simulink library "xps_library"  (Simulink 8.0)
settings: Solver=ode45  SolverMode=SingleTasking  StartTime=0.0  StopTime=10.0  RelTol=1e-3
undefined symbols (not defined in the file): sys_clk, xps_library_software_register_user_data_in
libraries: xbsIndex_r4 x867, simulink x109, dspsigops x81, casper_library_flow_control x68, xps_library x18, casper_library_misc x11
(part 3 of 10)

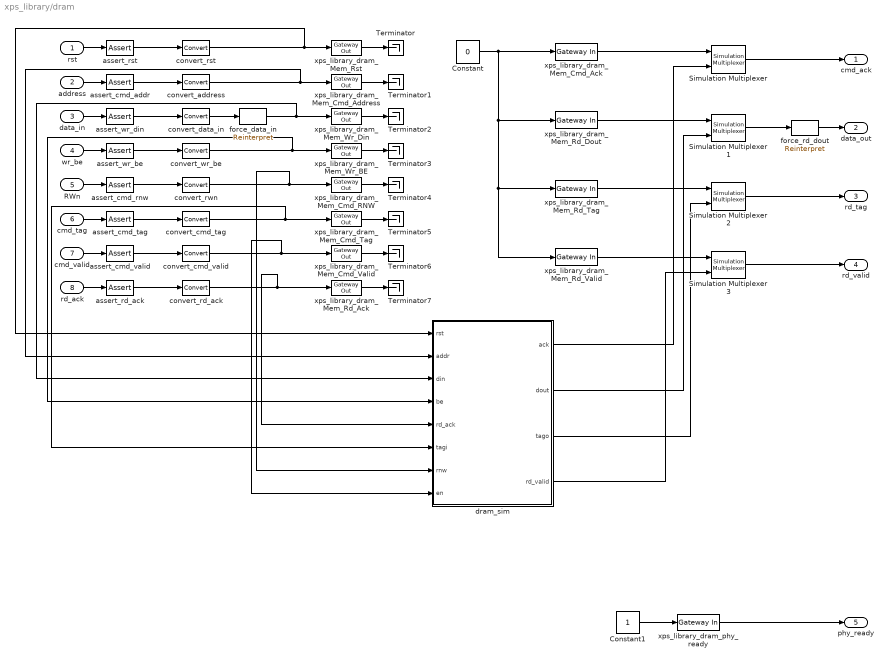
== system xps_library/dram ==
  rst : Inport
  address : Inport  Port=2
  data_in : Inport  Port=3
  wr_be : Inport  Port=4
  RWn : Inport  Port=5
  cmd_tag : Inport  Port=6
  cmd_valid : Inport  Port=7
  rd_ack : Inport  Port=8
  Constant : Constant  Value=0
  Constant1 : Constant
  Simulation Multiplexer{,1..3} (4 alike) : xbsIndex_r4/Simulation Multiplexer  sim_sel=2  hw_sel=1  block_type=simmux
      settings: infoedit="Distinguish input subsystems as \"simulation only\" and \"generation only\".  The input specified For Simulation will be used during Simulink simulation.  The input specified For Generation will be used during code generation.  This block will typically be used on the output of a HW Co-Simulation, Black Box, or ModelSim subsystem.<P><P>Hardware Notes: This block costs nothing."  block_version=9.1.01
  Terminator{,1..7} (8 alike) : Terminator
  assert_cmd_addr : xbsIndex_r4/Assert  assert_type=off  type_source=Explicitly  gui_display_data_type=Fixed-point  arith_type="Signed  (2's comp)"  n_bits=16  bin_pt=14  preci_type=Single  exp_width=8  frac_width=24  assert_rate=on  rate_source=Explicitly  period=sample_period  output_port=on  block_type=assert
      settings: infoedit=Asserts a user-defined sample rate and/or type on a signal.<P><P>Hardware notes: In hardware this block costs nothing.  block_version=9.1.01
  assert_cmd_rnw : xbsIndex_r4/Assert  assert_type=off  type_source=Explicitly  gui_display_data_type=Fixed-point  arith_type="Signed  (2's comp)"  n_bits=16  bin_pt=14  preci_type=Single  exp_width=8  frac_width=24  assert_rate=on  rate_source=Explicitly  period=sample_period  output_port=on  block_type=assert
      settings: infoedit=Asserts a user-defined sample rate and/or type on a signal.<P><P>Hardware notes: In hardware this block costs nothing.  block_version=9.1.01
  assert_cmd_tag : xbsIndex_r4/Assert  assert_type=off  type_source=Explicitly  gui_display_data_type=Fixed-point  arith_type="Signed  (2's comp)"  n_bits=16  bin_pt=14  preci_type=Single  exp_width=8  frac_width=24  assert_rate=on  rate_source=Explicitly  period=sample_period  output_port=on  block_type=assert
      settings: infoedit=Asserts a user-defined sample rate and/or type on a signal.<P><P>Hardware notes: In hardware this block costs nothing.  block_version=9.1.01
  assert_cmd_valid : xbsIndex_r4/Assert  assert_type=off  type_source=Explicitly  gui_display_data_type=Fixed-point  arith_type="Signed  (2's comp)"  n_bits=16  bin_pt=14  preci_type=Single  exp_width=8  frac_width=24  assert_rate=on  rate_source=Explicitly  period=sample_period  output_port=on  block_type=assert
      settings: infoedit=Asserts a user-defined sample rate and/or type on a signal.<P><P>Hardware notes: In hardware this block costs nothing.  block_version=9.1.01
  assert_rd_ack : xbsIndex_r4/Assert  assert_type=off  type_source=Explicitly  gui_display_data_type=Fixed-point  arith_type="Signed  (2's comp)"  n_bits=16  bin_pt=14  preci_type=Single  exp_width=8  frac_width=24  assert_rate=on  rate_source=Explicitly  period=sample_period  output_port=on  block_type=assert
      settings: infoedit=Asserts a user-defined sample rate and/or type on a signal.<P><P>Hardware notes: In hardware this block costs nothing.  block_version=9.1.01
  assert_rst : xbsIndex_r4/Assert  assert_type=off  type_source=Explicitly  gui_display_data_type=Fixed-point  arith_type="Signed  (2's comp)"  n_bits=16  bin_pt=14  preci_type=Single  exp_width=8  frac_width=24  assert_rate=on  rate_source=Explicitly  period=sample_period  output_port=on  block_type=assert
      settings: infoedit=Asserts a user-defined sample rate and/or type on a signal.<P><P>Hardware notes: In hardware this block costs nothing.  block_version=9.1.01
  assert_wr_be : xbsIndex_r4/Assert  assert_type=off  type_source=Explicitly  gui_display_data_type=Fixed-point  arith_type="Signed  (2's comp)"  n_bits=16  bin_pt=14  preci_type=Single  exp_width=8  frac_width=24  assert_rate=on  rate_source=Explicitly  period=sample_period  output_port=on  block_type=assert
      settings: infoedit=Asserts a user-defined sample rate and/or type on a signal.<P><P>Hardware notes: In hardware this block costs nothing.  block_version=9.1.01
  assert_wr_din : xbsIndex_r4/Assert  assert_type=off  type_source=Explicitly  gui_display_data_type=Fixed-point  arith_type="Signed  (2's comp)"  n_bits=16  bin_pt=14  preci_type=Single  exp_width=8  frac_width=24  assert_rate=on  rate_source=Explicitly  period=sample_period  output_port=on  block_type=assert
      settings: infoedit=Asserts a user-defined sample rate and/or type on a signal.<P><P>Hardware notes: In hardware this block costs nothing.  block_version=9.1.01
  convert_address : xbsIndex_r4/Convert  gui_display_data_type=Fixed-point  arith_type=Unsigned  n_bits=32  bin_pt=0  float_type=Single  exp_bits=8  fraction_bits=24  quantization=Truncate  overflow=Wrap  en=off  latency=0  dbl_ovrd=off  pipeline=off  block_type=convert
      settings: xl_area=[0, 0, 0, 0, 0, 0, 0]
  convert_cmd_tag : xbsIndex_r4/Convert  gui_display_data_type=Fixed-point  arith_type=Unsigned  n_bits=32  bin_pt=0  float_type=Single  exp_bits=8  fraction_bits=24  quantization=Truncate  overflow=Wrap  en=off  latency=0  dbl_ovrd=off  pipeline=off  block_type=convert
      settings: xl_area=[0, 0, 0, 0, 0, 0, 0]
  convert_cmd_valid : xbsIndex_r4/Convert  gui_display_data_type=Fixed-point  arith_type=Unsigned  n_bits=1  bin_pt=0  float_type=Single  exp_bits=8  fraction_bits=24  quantization=Truncate  overflow=Wrap  en=off  latency=0  dbl_ovrd=off  pipeline=off  block_type=convert
      settings: xl_area=[0, 0, 0, 0, 0, 0, 0]
  convert_data_in : xbsIndex_r4/Convert  gui_display_data_type=Fixed-point  arith_type=Unsigned  n_bits=144  bin_pt=0  float_type=Single  exp_bits=8  fraction_bits=24  quantization=Truncate  overflow=Wrap  en=off  latency=0  dbl_ovrd=off  pipeline=off  block_type=convert
      settings: xl_area=[0, 0, 0, 0, 0, 0, 0]
  convert_rd_ack : xbsIndex_r4/Convert  gui_display_data_type=Fixed-point  arith_type=Unsigned  n_bits=1  bin_pt=0  float_type=Single  exp_bits=8  fraction_bits=24  quantization=Truncate  overflow=Wrap  en=off  latency=0  dbl_ovrd=off  pipeline=off  block_type=convert
      settings: xl_area=[0, 0, 0, 0, 0, 0, 0]
  convert_rst : xbsIndex_r4/Convert  gui_display_data_type=Fixed-point  arith_type=Unsigned  n_bits=1  bin_pt=0  float_type=Single  exp_bits=8  fraction_bits=24  quantization=Truncate  overflow=Wrap  en=off  latency=0  dbl_ovrd=off  pipeline=off  block_type=convert
      settings: xl_area=[0, 0, 0, 0, 0, 0, 0]
  convert_rwn : xbsIndex_r4/Convert  gui_display_data_type=Fixed-point  arith_type=Unsigned  n_bits=1  bin_pt=0  float_type=Single  exp_bits=8  fraction_bits=24  quantization=Truncate  overflow=Wrap  en=off  latency=0  dbl_ovrd=off  pipeline=off  block_type=convert
      settings: xl_area=[0, 0, 0, 0, 0, 0, 0]
  convert_wr_be : xbsIndex_r4/Convert  gui_display_data_type=Fixed-point  arith_type=Unsigned  n_bits=18  bin_pt=0  float_type=Single  exp_bits=8  fraction_bits=24  quantization=Truncate  overflow=Wrap  en=off  latency=0  dbl_ovrd=off  pipeline=off  block_type=convert
      settings: xl_area=[0, 0, 0, 0, 0, 0, 0]
  dram_sim : Subsystem
  force_data_in : xbsIndex_r4/Reinterpret  force_arith_type=on  arith_type=Unsigned  force_bin_pt=on  bin_pt=0  block_type=reinterpret
      settings: infoedit="Changes signal type without altering the binary representation.   You can changed the signal between signed and unsigned, and relocate the binary point.<P><P>Hardware notes: In hardware this block costs nothing.<P><P>Example:  Suppose the input is 6 bits wide, signed, with 2 fractional bits, and the output is forced to unsigned with 0 fractional bits.  Then an input of -2.0 (1110.00 in binary 2's complement) becomes an output of 56 (111000 in binary)."  block_version=9.1.01
  force_rd_dout : xbsIndex_r4/Reinterpret  force_arith_type=on  arith_type=Unsigned  force_bin_pt=on  bin_pt=0  block_type=reinterpret
      settings: infoedit="Changes signal type without altering the binary representation.   You can changed the signal between signed and unsigned, and relocate the binary point.<P><P>Hardware notes: In hardware this block costs nothing.<P><P>Example:  Suppose the input is 6 bits wide, signed, with 2 fractional bits, and the output is forced to unsigned with 0 fractional bits.  Then an input of -2.0 (1110.00 in binary 2's complement) becomes an output of 56 (111000 in binary)."  block_version=9.1.01
  xps_library_dram_Mem_Cmd_Ack : xbsIndex_r4/Gateway In  gui_display_data_type=Fixed-point  arith_type=Boolean  n_bits=1  bin_pt=0  preci_type=Single  exp_width=8  frac_width=24  quantization=Truncate  overflow=Wrap  period=sample_period  dbl_ovrd=off  timing_constraint=None  locs_specified=off  LOCs={}  hdl_port=on  block_type=gatewayin
      settings: infoedit="Gateway in block.  Converts inputs of type Simulink integer, double and fixed point to  Xilinx fixed point type.<P><P>Hardware notes:  In hardware these blocks become top level input ports."  xl_area=[0, 0, 0, 0, 0, 0, 0]
  xps_library_dram_Mem_Cmd_Address : xbsIndex_r4/Gateway Out  hdl_port=on  timing_constraint=None  locs_specified=off  LOCs={}  block_type=gatewayout
      settings: infoedit="Gateway out block.  Converts Xilinx fixed point inputs into ouputs of type Simulink integer, double, or fixed point.<P><P>Hardware notes:  In hardware these blocks become top level output ports or are discarded, depending on how they are configured."  xl_area=[0, 0, 0, 0, 0, 0, 0]
  xps_library_dram_Mem_Cmd_RNW : xbsIndex_r4/Gateway Out  hdl_port=on  timing_constraint=None  locs_specified=off  LOCs={}  block_type=gatewayout
      settings: infoedit="Gateway out block.  Converts Xilinx fixed point inputs into ouputs of type Simulink integer, double, or fixed point.<P><P>Hardware notes:  In hardware these blocks become top level output ports or are discarded, depending on how they are configured."  xl_area=[0, 0, 0, 0, 0, 0, 0]
  xps_library_dram_Mem_Cmd_Tag : xbsIndex_r4/Gateway Out  hdl_port=on  timing_constraint=None  locs_specified=off  LOCs={}  block_type=gatewayout
      settings: infoedit="Gateway out block.  Converts Xilinx fixed point inputs into ouputs of type Simulink integer, double, or fixed point.<P><P>Hardware notes:  In hardware these blocks become top level output ports or are discarded, depending on how they are configured."  xl_area=[0, 0, 0, 0, 0, 0, 0]
  xps_library_dram_Mem_Cmd_Valid : xbsIndex_r4/Gateway Out  hdl_port=on  timing_constraint=None  locs_specified=off  LOCs={}  block_type=gatewayout
      settings: infoedit="Gateway out block.  Converts Xilinx fixed point inputs into ouputs of type Simulink integer, double, or fixed point.<P><P>Hardware notes:  In hardware these blocks become top level output ports or are discarded, depending on how they are configured."  xl_area=[0, 0, 0, 0, 0, 0, 0]
  xps_library_dram_Mem_Rd_Ack : xbsIndex_r4/Gateway Out  hdl_port=on  timing_constraint=None  locs_specified=off  LOCs={}  block_type=gatewayout
      settings: infoedit="Gateway out block.  Converts Xilinx fixed point inputs into ouputs of type Simulink integer, double, or fixed point.<P><P>Hardware notes:  In hardware these blocks become top level output ports or are discarded, depending on how they are configured."  xl_area=[0, 0, 0, 0, 0, 0, 0]
  xps_library_dram_Mem_Rd_Dout : xbsIndex_r4/Gateway In  gui_display_data_type=Fixed-point  arith_type=Unsigned  n_bits=144  bin_pt=0  preci_type=Single  exp_width=8  frac_width=24  quantization=Truncate  overflow=Wrap  period=sample_period  dbl_ovrd=off  timing_constraint=None  locs_specified=off  LOCs={}  hdl_port=on  block_type=gatewayin
      settings: infoedit="Gateway in block.  Converts inputs of type Simulink integer, double and fixed point to  Xilinx fixed point type.<P><P>Hardware notes:  In hardware these blocks become top level input ports."  xl_area=[0, 0, 0, 0, 0, 0, 0]
  xps_library_dram_Mem_Rd_Tag : xbsIndex_r4/Gateway In  gui_display_data_type=Fixed-point  arith_type=Unsigned  n_bits=32  bin_pt=0  preci_type=Single  exp_width=8  frac_width=24  quantization=Truncate  overflow=Wrap  period=sample_period  dbl_ovrd=off  timing_constraint=None  locs_specified=off  LOCs={}  hdl_port=on  block_type=gatewayin
      settings: infoedit="Gateway in block.  Converts inputs of type Simulink integer, double and fixed point to  Xilinx fixed point type.<P><P>Hardware notes:  In hardware these blocks become top level input ports."  xl_area=[0, 0, 0, 0, 0, 0, 0]
  xps_library_dram_Mem_Rd_Valid : xbsIndex_r4/Gateway In  gui_display_data_type=Fixed-point  arith_type=Boolean  n_bits=1  bin_pt=0  preci_type=Single  exp_width=8  frac_width=24  quantization=Truncate  overflow=Wrap  period=sample_period  dbl_ovrd=off  timing_constraint=None  locs_specified=off  LOCs={}  hdl_port=on  block_type=gatewayin
      settings: infoedit="Gateway in block.  Converts inputs of type Simulink integer, double and fixed point to  Xilinx fixed point type.<P><P>Hardware notes:  In hardware these blocks become top level input ports."  xl_area=[0, 0, 0, 0, 0, 0, 0]
  xps_library_dram_Mem_Rst : xbsIndex_r4/Gateway Out  hdl_port=on  timing_constraint=None  locs_specified=off  LOCs={}  block_type=gatewayout
      settings: infoedit="Gateway out block.  Converts Xilinx fixed point inputs into ouputs of type Simulink integer, double, or fixed point.<P><P>Hardware notes:  In hardware these blocks become top level output ports or are discarded, depending on how they are configured."  xl_area=[0, 0, 0, 0, 0, 0, 0]
  xps_library_dram_Mem_Wr_BE : xbsIndex_r4/Gateway Out  hdl_port=on  timing_constraint=None  locs_specified=off  LOCs={}  block_type=gatewayout
      settings: infoedit="Gateway out block.  Converts Xilinx fixed point inputs into ouputs of type Simulink integer, double, or fixed point.<P><P>Hardware notes:  In hardware these blocks become top level output ports or are discarded, depending on how they are configured."  xl_area=[0, 0, 0, 0, 0, 0, 0]
  xps_library_dram_Mem_Wr_Din : xbsIndex_r4/Gateway Out  hdl_port=on  timing_constraint=None  locs_specified=off  LOCs={}  block_type=gatewayout
      settings: infoedit="Gateway out block.  Converts Xilinx fixed point inputs into ouputs of type Simulink integer, double, or fixed point.<P><P>Hardware notes:  In hardware these blocks become top level output ports or are discarded, depending on how they are configured."  xl_area=[0, 0, 0, 0, 0, 0, 0]
  xps_library_dram_phy_ready : xbsIndex_r4/Gateway In  gui_display_data_type=Fixed-point  arith_type=Boolean  n_bits=1  bin_pt=0  preci_type=Single  exp_width=8  frac_width=24  quantization=Truncate  overflow=Wrap  period=sample_period  dbl_ovrd=off  timing_constraint=None  locs_specified=off  LOCs={}  hdl_port=on  block_type=gatewayin
      settings: infoedit="Gateway in block.  Converts inputs of type Simulink integer, double and fixed point to  Xilinx fixed point type.<P><P>Hardware notes:  In hardware these blocks become top level input ports."  xl_area=[0, 0, 0, 0, 0, 0, 0]
  cmd_ack : Outport
  data_out : Outport  Port=2
  rd_tag : Outport  Port=3
  rd_valid : Outport  Port=4
  phy_ready : Outport  Port=5
  wires:
  Constant1/1 -> xps_library_dram_phy_ready/1
  xps_library_dram_phy_ready/1 -> phy_ready/1
  dram_sim/4(rd_valid) -> Simulation Multiplexer3/2
  dram_sim/3(tago) -> Simulation Multiplexer2/2
  dram_sim/2(dout) -> Simulation Multiplexer1/2
  dram_sim/1(ack) -> Simulation Multiplexer/2
  xps_library_dram_Mem_Rd_Valid/1 -> Simulation Multiplexer3/1
  xps_library_dram_Mem_Rd_Tag/1 -> Simulation Multiplexer2/1
  Simulation Multiplexer3/1 -> rd_valid/1
  Simulation Multiplexer2/1 -> rd_tag/1
  Simulation Multiplexer1/1 -> force_rd_dout/1
  xps_library_dram_Mem_Rd_Dout/1 -> Simulation Multiplexer1/1
  Simulation Multiplexer/1 -> cmd_ack/1
  xps_library_dram_Mem_Cmd_Ack/1 -> Simulation Multiplexer/1
  Constant/1 -> xps_library_dram_Mem_Rd_Valid/1, xps_library_dram_Mem_Rd_Tag/1, xps_library_dram_Mem_Rd_Dout/1, xps_library_dram_Mem_Cmd_Ack/1
  xps_library_dram_Mem_Rd_Ack/1 -> Terminator7/1
  xps_library_dram_Mem_Cmd_Valid/1 -> Terminator6/1
  xps_library_dram_Mem_Cmd_Tag/1 -> Terminator5/1
  xps_library_dram_Mem_Cmd_RNW/1 -> Terminator4/1
  xps_library_dram_Mem_Wr_BE/1 -> Terminator3/1
  xps_library_dram_Mem_Wr_Din/1 -> Terminator2/1
  xps_library_dram_Mem_Cmd_Address/1 -> Terminator1/1
  xps_library_dram_Mem_Rst/1 -> Terminator/1
  force_data_in/1 -> xps_library_dram_Mem_Wr_Din/1, dram_sim/3(din)
  force_rd_dout/1 -> data_out/1
  assert_rst/1 -> convert_rst/1
  assert_cmd_addr/1 -> convert_address/1
  assert_wr_din/1 -> convert_data_in/1
  assert_wr_be/1 -> convert_wr_be/1
  assert_cmd_rnw/1 -> convert_rwn/1
  assert_cmd_tag/1 -> convert_cmd_tag/1
  assert_cmd_valid/1 -> convert_cmd_valid/1
  assert_rd_ack/1 -> convert_rd_ack/1
  rst/1 -> assert_rst/1
  address/1 -> assert_cmd_addr/1
  data_in/1 -> assert_wr_din/1
  wr_be/1 -> assert_wr_be/1
  RWn/1 -> assert_cmd_rnw/1
  cmd_tag/1 -> assert_cmd_tag/1
  cmd_valid/1 -> assert_cmd_valid/1
  rd_ack/1 -> assert_rd_ack/1
  convert_rst/1 -> xps_library_dram_Mem_Rst/1, dram_sim/1(rst)
  convert_address/1 -> xps_library_dram_Mem_Cmd_Address/1, dram_sim/2(addr)
  convert_data_in/1 -> force_data_in/1
  convert_wr_be/1 -> xps_library_dram_Mem_Wr_BE/1, dram_sim/4(be)
  convert_rwn/1 -> xps_library_dram_Mem_Cmd_RNW/1, dram_sim/7(rnw)
  convert_cmd_tag/1 -> xps_library_dram_Mem_Cmd_Tag/1, dram_sim/6(tagi)
  convert_cmd_valid/1 -> xps_library_dram_Mem_Cmd_Valid/1, dram_sim/8(en)
  convert_rd_ack/1 -> xps_library_dram_Mem_Rd_Ack/1, dram_sim/5(rd_ack)

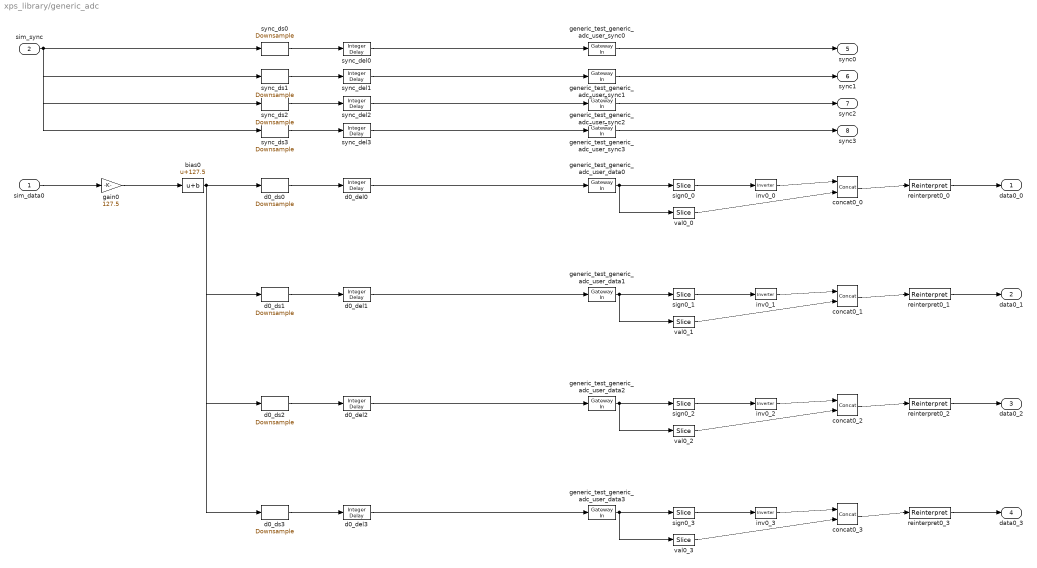
== system xps_library/generic_adc ==
  sim_data0 : Inport
  sim_sync : Inport  Port=2
  bias0 : Bias  Bias=127.5  SaturateOnIntegerOverflow=on
  concat0_{0..3} (4 alike) : xbsIndex_r4/Concat  num_inputs=2  dbl_ovrd=off  block_type=concat
  d0_del0 : simulink/Discrete/Integer Delay  NumDelays=2  vinit=0.0  samptime=-1
  d0_del1 : simulink/Discrete/Integer Delay  NumDelays=1  vinit=0.0  samptime=-1
  d0_del2 : simulink/Discrete/Integer Delay  NumDelays=1  vinit=0.0  samptime=-1
  d0_del3 : simulink/Discrete/Integer Delay  NumDelays=1  vinit=0.0  samptime=-1
  d0_ds0 : dspsigops/Downsample  N=4  phase=0  smode=Force single rate  fmode=Maintain input frame rate  ic=0
  d0_ds1 : dspsigops/Downsample  N=4  phase=1  smode=Force single rate  fmode=Maintain input frame rate  ic=0
  d0_ds2 : dspsigops/Downsample  N=4  phase=2  smode=Force single rate  fmode=Maintain input frame rate  ic=0
  d0_ds3 : dspsigops/Downsample  N=4  phase=3  smode=Force single rate  fmode=Maintain input frame rate  ic=0
  gain0 : Gain  Gain=127.5  SaturateOnIntegerOverflow=on  OutDataTypeStr=Inherit: Same as input  ParamDataTypeStr=Inherit: Same as input
  generic_test_generic_adc_user_data{0..3} (4 alike) : xbsIndex_r4/Gateway In  gui_display_data_type=Fixed-point  arith_type="Signed  (2's comp)"  n_bits=8  bin_pt=0  preci_type=Single  exp_width=8  frac_width=24  quantization="Round  (unbiased: +/- Inf)"  overflow=Saturate  period=1  dbl_ovrd=off  timing_constraint=None  locs_specified=off  LOCs={}  hdl_port=on  block_type=gatewayin
      settings: infoedit="Gateway in block.  Converts inputs of type Simulink integer, double and fixed point to  Xilinx fixed point type.<br><br>Hardware notes:  In hardware these blocks become top level input ports."  block_version=11.4
  generic_test_generic_adc_user_sync{0..3} (4 alike) : xbsIndex_r4/Gateway In  gui_display_data_type=Fixed-point  arith_type=Boolean  n_bits=16  bin_pt=14  preci_type=Single  exp_width=8  frac_width=24  quantization="Round  (unbiased: +/- Inf)"  overflow=Saturate  period=1  dbl_ovrd=off  timing_constraint=None  locs_specified=off  LOCs={}  hdl_port=on  block_type=gatewayin
      settings: infoedit="Gateway in block.  Converts inputs of type Simulink integer, double and fixed point to  Xilinx fixed point type.<br><br>Hardware notes:  In hardware these blocks become top level input ports."  block_version=11.4
  inv0_{0..3} (4 alike) : xbsIndex_r4/Inverter  en=off  latency=0  dbl_ovrd=off  block_type=inv
      settings: block_version=11.4
  reinterpret0_{0..3} (4 alike) : xbsIndex_r4/Reinterpret  force_arith_type=on  arith_type="Signed  (2's comp)"  force_bin_pt=on  bin_pt=7  block_type=reinterpret
      settings: infoedit="Changes signal type without altering the binary representation.   You can changed the signal between signed and unsigned, and relocate the binary point.<br><br>Hardware notes: In hardware this block costs nothing.<br><br>Example:  Suppose the input is 6 bits wide, signed, with 2 fractional bits, and the output is forced to unsigned with 0 fractional bits.  Then an input of -2.0 (1110.00 in binary 2's complement) becomes an output of 56 (111000 in binary)."
  sign0_{0..3} (4 alike) : xbsIndex_r4/Slice  nbits=1  boolean_output=off  mode=Upper Bit Location + Width  bit1=0  base1=MSB of Input  bit0=0  base0=MSB of Input  dbl_ovrd=off  block_type=slice
  sync_del0 : simulink/Discrete/Integer Delay  NumDelays=2  vinit=0.0  samptime=-1
  sync_del1 : simulink/Discrete/Integer Delay  NumDelays=1  vinit=0.0  samptime=-1
  sync_del2 : simulink/Discrete/Integer Delay  NumDelays=1  vinit=0.0  samptime=-1
  sync_del3 : simulink/Discrete/Integer Delay  NumDelays=1  vinit=0.0  samptime=-1
  sync_ds0 : dspsigops/Downsample  N=4  phase=0  smode=Force single rate  fmode=Maintain input frame rate  ic=0
  sync_ds1 : dspsigops/Downsample  N=4  phase=1  smode=Force single rate  fmode=Maintain input frame rate  ic=0
  sync_ds2 : dspsigops/Downsample  N=4  phase=2  smode=Force single rate  fmode=Maintain input frame rate  ic=0
  sync_ds3 : dspsigops/Downsample  N=4  phase=3  smode=Force single rate  fmode=Maintain input frame rate  ic=0
  val0_{0..3} (4 alike) : xbsIndex_r4/Slice  nbits=7  boolean_output=off  mode=Lower Bit Location + Width  bit1=0  base1=LSB of Input  bit0=0  base0=LSB of Input  dbl_ovrd=off  block_type=slice
  data0_0 : Outport
  data0_1 : Outport  Port=2
  data0_2 : Outport  Port=3
  data0_3 : Outport  Port=4
  sync0 : Outport  Port=5
  sync1 : Outport  Port=6
  sync2 : Outport  Port=7
  sync3 : Outport  Port=8
  wires:
  generic_test_generic_adc_user_sync3/1 -> sync3/1
  sync_del3/1 -> generic_test_generic_adc_user_sync3/1
  sync_ds3/1 -> sync_del3/1
  generic_test_generic_adc_user_sync2/1 -> sync2/1
  sync_del2/1 -> generic_test_generic_adc_user_sync2/1
  sync_ds2/1 -> sync_del2/1
  generic_test_generic_adc_user_sync1/1 -> sync1/1
  sync_del1/1 -> generic_test_generic_adc_user_sync1/1
  sync_ds1/1 -> sync_del1/1
  generic_test_generic_adc_user_sync0/1 -> sync0/1
  sync_del0/1 -> generic_test_generic_adc_user_sync0/1
  sync_ds0/1 -> sync_del0/1
  sim_sync/1 -> sync_ds3/1, sync_ds2/1, sync_ds1/1, sync_ds0/1
  reinterpret0_3/1 -> data0_3/1
  concat0_3/1 -> reinterpret0_3/1
  val0_3/1 -> concat0_3/2
  inv0_3/1 -> concat0_3/1
  sign0_3/1 -> inv0_3/1
  generic_test_generic_adc_user_data3/1 -> val0_3/1, sign0_3/1
  d0_del3/1 -> generic_test_generic_adc_user_data3/1
  d0_ds3/1 -> d0_del3/1
  reinterpret0_2/1 -> data0_2/1
  concat0_2/1 -> reinterpret0_2/1
  val0_2/1 -> concat0_2/2
  inv0_2/1 -> concat0_2/1
  sign0_2/1 -> inv0_2/1
  generic_test_generic_adc_user_data2/1 -> val0_2/1, sign0_2/1
  d0_del2/1 -> generic_test_generic_adc_user_data2/1
  d0_ds2/1 -> d0_del2/1
  reinterpret0_1/1 -> data0_1/1
  concat0_1/1 -> reinterpret0_1/1
  val0_1/1 -> concat0_1/2
  inv0_1/1 -> concat0_1/1
  sign0_1/1 -> inv0_1/1
  generic_test_generic_adc_user_data1/1 -> val0_1/1, sign0_1/1
  d0_del1/1 -> generic_test_generic_adc_user_data1/1
  d0_ds1/1 -> d0_del1/1
  reinterpret0_0/1 -> data0_0/1
  concat0_0/1 -> reinterpret0_0/1
  val0_0/1 -> concat0_0/2
  inv0_0/1 -> concat0_0/1
  sign0_0/1 -> inv0_0/1
  generic_test_generic_adc_user_data0/1 -> val0_0/1, sign0_0/1
  d0_del0/1 -> generic_test_generic_adc_user_data0/1
  d0_ds0/1 -> d0_del0/1
  bias0/1 -> d0_ds3/1, d0_ds2/1, d0_ds1/1, d0_ds0/1
  gain0/1 -> bias0/1
  sim_data0/1 -> gain0/1

== system xps_library/gpio ==
  gpio_out : Inport
  xps_library_gpio_gateway : xbsIndex_r4/Gateway Out  hdl_port=on  timing_constraint=None  locs_specified=off  LOCs={}  block_type=gatewayout
      settings: infoedit="Gateway out block.  Converts Xilinx fixed point or floating-point type inputs into ouputs of type Simulink integer, double, or fixed point.<br><br>Hardware notes:  In hardware these blocks become top level output ports or are discarded, depending on how they are configured."
  sim_out : Outport
  wires:
  xps_library_gpio_gateway/1 -> sim_out/1
  ? -> xps_library_gpio_gateway/1
  gpio_out/1 -> ?

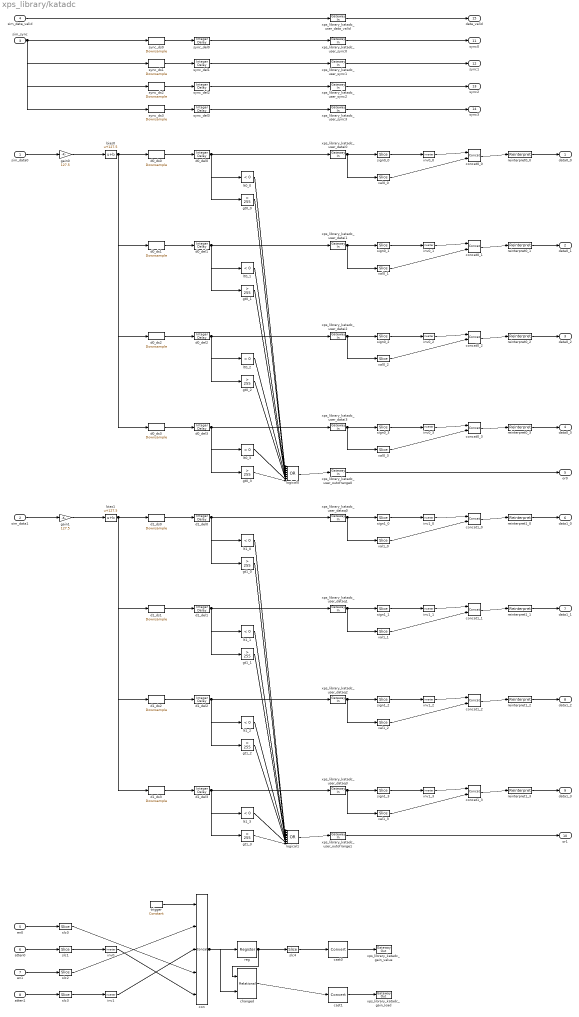
== system xps_library/katadc ==
  sim_data0 : Inport
  sim_data1 : Inport  Port=2
  sim_sync : Inport  Port=3
  sim_data_valid : Inport  Port=4
  en0 : Inport  Port=5
  atten0 : Inport  Port=6
  en1 : Inport  Port=7
  atten1 : Inport  Port=8
  bias0 : Bias  Bias=127.5  SaturateOnIntegerOverflow=on
  bias1 : Bias  Bias=127.5  SaturateOnIntegerOverflow=on
  cast0 : xbsIndex_r4/Convert  gui_display_data_type=Fixed-point  arith_type=Unsigned  n_bits=14  bin_pt=0  float_type=Single  exp_bits=8  fraction_bits=24  quantization=Truncate  overflow=Wrap  en=off  latency=0  dbl_ovrd=off  pipeline=off  block_type=convert
      settings: block_version=11.4
  cast1 : xbsIndex_r4/Convert  gui_display_data_type=Fixed-point  arith_type=Boolean  n_bits=16  bin_pt=14  float_type=Single  exp_bits=8  fraction_bits=24  quantization=Truncate  overflow=Wrap  en=off  latency=0  dbl_ovrd=off  pipeline=off  block_type=convert
      settings: block_version=11.4
  changed : xbsIndex_r4/Relational  mode=a!=b  en=off  latency=1  dbl_ovrd=off  block_type=relational
  con : xbsIndex_r4/Concat  num_inputs=5  dbl_ovrd=off  block_type=concat
  concat0_{0..3} (4 alike) : xbsIndex_r4/Concat  num_inputs=2  dbl_ovrd=off  block_type=concat
  concat1_{0..3} (4 alike) : xbsIndex_r4/Concat  num_inputs=2  dbl_ovrd=off  block_type=concat
  d0_del0 : simulink/Discrete/Integer Delay  NumDelays=2  vinit=0.0  samptime=-1
  d0_del1 : simulink/Discrete/Integer Delay  NumDelays=1  vinit=0.0  samptime=-1
  d0_del2 : simulink/Discrete/Integer Delay  NumDelays=1  vinit=0.0  samptime=-1
  d0_del3 : simulink/Discrete/Integer Delay  NumDelays=1  vinit=0.0  samptime=-1
  d0_ds0 : dspsigops/Downsample  N=4  phase=0  smode=Allow multirate  fmode=Maintain input frame size  ic=0
  d0_ds1 : dspsigops/Downsample  N=4  phase=1  smode=Allow multirate  fmode=Maintain input frame size  ic=0
  d0_ds2 : dspsigops/Downsample  N=4  phase=2  smode=Allow multirate  fmode=Maintain input frame size  ic=0
  d0_ds3 : dspsigops/Downsample  N=4  phase=3  smode=Allow multirate  fmode=Maintain input frame size  ic=0
  d1_del0 : simulink/Discrete/Integer Delay  NumDelays=2  vinit=0.0  samptime=-1
  d1_del1 : simulink/Discrete/Integer Delay  NumDelays=1  vinit=0.0  samptime=-1
  d1_del2 : simulink/Discrete/Integer Delay  NumDelays=1  vinit=0.0  samptime=-1
  d1_del3 : simulink/Discrete/Integer Delay  NumDelays=1  vinit=0.0  samptime=-1
  d1_ds0 : dspsigops/Downsample  N=4  phase=0  smode=Allow multirate  fmode=Maintain input frame size  ic=0
  d1_ds1 : dspsigops/Downsample  N=4  phase=1  smode=Allow multirate  fmode=Maintain input frame size  ic=0
  d1_ds2 : dspsigops/Downsample  N=4  phase=2  smode=Allow multirate  fmode=Maintain input frame size  ic=0
  d1_ds3 : dspsigops/Downsample  N=4  phase=3  smode=Allow multirate  fmode=Maintain input frame size  ic=0
  gain0 : Gain  Gain=127.5  SaturateOnIntegerOverflow=on  OutDataTypeStr=Inherit: Same as input  ParamDataTypeStr=Inherit: Same as input
  gain1 : Gain  Gain=127.5  SaturateOnIntegerOverflow=on  OutDataTypeStr=Inherit: Same as input  ParamDataTypeStr=Inherit: Same as input
  gt0_{0..3} (4 alike) : simulink/Logic and Bit Operations/Compare To Constant  relop=>  const=255  LogicOutDataTypeMode=boolean  ZeroCross=off
  gt1_{0..3} (4 alike) : simulink/Logic and Bit Operations/Compare To Constant  relop=>  const=255  LogicOutDataTypeMode=boolean  ZeroCross=off
  inv0 : xbsIndex_r4/Inverter  en=off  latency=0  dbl_ovrd=off  block_type=inv
      settings: block_version=11.4
  inv0_{0..3} (4 alike) : xbsIndex_r4/Inverter  en=off  latency=0  dbl_ovrd=off  block_type=inv
      settings: block_version=11.4
  inv1 : xbsIndex_r4/Inverter  en=off  latency=0  dbl_ovrd=off  block_type=inv
      settings: block_version=11.4
  inv1_{0..3} (4 alike) : xbsIndex_r4/Inverter  en=off  latency=0  dbl_ovrd=off  block_type=inv
      settings: block_version=11.4
  logical0 : Logic  Operator=OR  Inputs=8
  logical1 : Logic  Operator=OR  Inputs=8
  lt0_{0..3} (4 alike) : simulink/Logic and Bit Operations/Compare To Constant  relop=<  const=0  LogicOutDataTypeMode=boolean  ZeroCross=off
  lt1_{0..3} (4 alike) : simulink/Logic and Bit Operations/Compare To Constant  relop=<  const=0  LogicOutDataTypeMode=boolean  ZeroCross=off
  reg : xbsIndex_r4/Register  init=0  rst=off  en=off  dbl_ovrd=off  block_type=register
      settings: block_version=11.4
  reinterpret0_{0..3} (4 alike) : xbsIndex_r4/Reinterpret  force_arith_type=on  arith_type="Signed  (2's comp)"  force_bin_pt=on  bin_pt=7  block_type=reinterpret
      settings: infoedit="Changes signal type without altering the binary representation.   You can changed the signal between signed and unsigned, and relocate the binary point.<br><br>Hardware notes: In hardware this block costs nothing.<br><br>Example:  Suppose the input is 6 bits wide, signed, with 2 fractional bits, and the output is forced to unsigned with 0 fractional bits.  Then an input of -2.0 (1110.00 in binary 2's complement) becomes an output of 56 (111000 in binary)."
  reinterpret1_{0..3} (4 alike) : xbsIndex_r4/Reinterpret  force_arith_type=on  arith_type="Signed  (2's comp)"  force_bin_pt=on  bin_pt=7  block_type=reinterpret
      settings: infoedit="Changes signal type without altering the binary representation.   You can changed the signal between signed and unsigned, and relocate the binary point.<br><br>Hardware notes: In hardware this block costs nothing.<br><br>Example:  Suppose the input is 6 bits wide, signed, with 2 fractional bits, and the output is forced to unsigned with 0 fractional bits.  Then an input of -2.0 (1110.00 in binary 2's complement) becomes an output of 56 (111000 in binary)."
  sign0_{0..3} (4 alike) : xbsIndex_r4/Slice  nbits=1  boolean_output=off  mode=Upper Bit Location + Width  bit1=0  base1=MSB of Input  bit0=0  base0=MSB of Input  dbl_ovrd=off  block_type=slice
  sign1_{0..3} (4 alike) : xbsIndex_r4/Slice  nbits=1  boolean_output=off  mode=Upper Bit Location + Width  bit1=0  base1=MSB of Input  bit0=0  base0=MSB of Input  dbl_ovrd=off  block_type=slice
  slc0 : xbsIndex_r4/Slice  nbits=1  boolean_output=off  mode=Lower Bit Location + Width  bit1=0  base1=MSB of Input  bit0=0  base0=LSB of Input  dbl_ovrd=off  block_type=slice
  slc1 : xbsIndex_r4/Slice  nbits=6  boolean_output=off  mode=Lower Bit Location + Width  bit1=0  base1=MSB of Input  bit0=0  base0=LSB of Input  dbl_ovrd=off  block_type=slice
  slc2 : xbsIndex_r4/Slice  nbits=1  boolean_output=off  mode=Lower Bit Location + Width  bit1=0  base1=MSB of Input  bit0=0  base0=LSB of Input  dbl_ovrd=off  block_type=slice
  slc3 : xbsIndex_r4/Slice  nbits=6  boolean_output=off  mode=Lower Bit Location + Width  bit1=0  base1=MSB of Input  bit0=0  base0=LSB of Input  dbl_ovrd=off  block_type=slice
  slc4 : xbsIndex_r4/Slice  nbits=14  boolean_output=off  mode=Lower Bit Location + Width  bit1=0  base1=MSB of Input  bit0=0  base0=LSB of Input  dbl_ovrd=off  block_type=slice
  sync_del0 : simulink/Discrete/Integer Delay  NumDelays=2  vinit=0.0  samptime=-1
  sync_del1 : simulink/Discrete/Integer Delay  NumDelays=1  vinit=0.0  samptime=-1
  sync_del2 : simulink/Discrete/Integer Delay  NumDelays=1  vinit=0.0  samptime=-1
  sync_del3 : simulink/Discrete/Integer Delay  NumDelays=1  vinit=0.0  samptime=-1
  sync_ds0 : dspsigops/Downsample  N=4  phase=0  smode=Allow multirate  fmode=Maintain input frame size  ic=0
  sync_ds1 : dspsigops/Downsample  N=4  phase=1  smode=Allow multirate  fmode=Maintain input frame size  ic=0
  sync_ds2 : dspsigops/Downsample  N=4  phase=2  smode=Allow multirate  fmode=Maintain input frame size  ic=0
  sync_ds3 : dspsigops/Downsample  N=4  phase=3  smode=Allow multirate  fmode=Maintain input frame size  ic=0
  trigger : xbsIndex_r4/Constant  const=1  gui_display_data_type=Fixed-point  arith_type=Unsigned  n_bits=1  bin_pt=0  preci_type=Single  exp_width=8  frac_width=24  explicit_period=off  period=1  equ=P=C  opselect=C  inp2=PCIN>>17  opr=+  inp1=P  carry=CIN  dbl_ovrd=off  block_type=constant
      settings: block_version=11.4
  val0_{0..3} (4 alike) : xbsIndex_r4/Slice  nbits=7  boolean_output=off  mode=Lower Bit Location + Width  bit1=0  base1=LSB of Input  bit0=0  base0=LSB of Input  dbl_ovrd=off  block_type=slice
  val1_{0..3} (4 alike) : xbsIndex_r4/Slice  nbits=7  boolean_output=off  mode=Lower Bit Location + Width  bit1=0  base1=LSB of Input  bit0=0  base0=LSB of Input  dbl_ovrd=off  block_type=slice
  xps_library_katadc_gain_load : xbsIndex_r4/Gateway Out  hdl_port=on  timing_constraint=None  locs_specified=off  LOCs={}  block_type=gatewayout
  xps_library_katadc_gain_value : xbsIndex_r4/Gateway Out  hdl_port=on  timing_constraint=None  locs_specified=off  LOCs={}  block_type=gatewayout
  xps_library_katadc_user_data_valid : xbsIndex_r4/Gateway In  gui_display_data_type=Fixed-point  arith_type=Boolean  n_bits=16  bin_pt=14  preci_type=Single  exp_width=8  frac_width=24  quantization="Round  (unbiased: +/- Inf)"  overflow=Saturate  period=1  dbl_ovrd=off  timing_constraint=None  locs_specified=off  LOCs={}  hdl_port=on  block_type=gatewayin
  xps_library_katadc_user_datai{0..3} (4 alike) : xbsIndex_r4/Gateway In  gui_display_data_type=Fixed-point  arith_type=Unsigned  n_bits=8  bin_pt=0  preci_type=Single  exp_width=8  frac_width=24  quantization="Round  (unbiased: +/- Inf)"  overflow=Saturate  period=1  dbl_ovrd=off  timing_constraint=None  locs_specified=off  LOCs={}  hdl_port=on  block_type=gatewayin
  xps_library_katadc_user_dataq{0..3} (4 alike) : xbsIndex_r4/Gateway In  gui_display_data_type=Fixed-point  arith_type=Unsigned  n_bits=8  bin_pt=0  preci_type=Single  exp_width=8  frac_width=24  quantization="Round  (unbiased: +/- Inf)"  overflow=Saturate  period=1  dbl_ovrd=off  timing_constraint=None  locs_specified=off  LOCs={}  hdl_port=on  block_type=gatewayin
  xps_library_katadc_user_outofrange0 : xbsIndex_r4/Gateway In  gui_display_data_type=Fixed-point  arith_type=Boolean  n_bits=16  bin_pt=14  preci_type=Single  exp_width=8  frac_width=24  quantization="Round  (unbiased: +/- Inf)"  overflow=Saturate  period=1  dbl_ovrd=off  timing_constraint=None  locs_specified=off  LOCs={}  hdl_port=on  block_type=gatewayin
  xps_library_katadc_user_outofrange1 : xbsIndex_r4/Gateway In  gui_display_data_type=Fixed-point  arith_type=Boolean  n_bits=16  bin_pt=14  preci_type=Single  exp_width=8  frac_width=24  quantization="Round  (unbiased: +/- Inf)"  overflow=Saturate  period=1  dbl_ovrd=off  timing_constraint=None  locs_specified=off  LOCs={}  hdl_port=on  block_type=gatewayin
  xps_library_katadc_user_sync{0..3} (4 alike) : xbsIndex_r4/Gateway In  gui_display_data_type=Fixed-point  arith_type=Boolean  n_bits=16  bin_pt=14  preci_type=Single  exp_width=8  frac_width=24  quantization="Round  (unbiased: +/- Inf)"  overflow=Saturate  period=1  dbl_ovrd=off  timing_constraint=None  locs_specified=off  LOCs={}  hdl_port=on  block_type=gatewayin
  data0_0 : Outport
  data0_1 : Outport  Port=2
  data0_2 : Outport  Port=3
  data0_3 : Outport  Port=4
  or0 : Outport  Port=5
  data1_0 : Outport  Port=6
  data1_1 : Outport  Port=7
  data1_2 : Outport  Port=8
  data1_3 : Outport  Port=9
  or1 : Outport  Port=10
  sync0 : Outport  Port=11
  sync1 : Outport  Port=12
  sync2 : Outport  Port=13
  sync3 : Outport  Port=14
  data_valid : Outport  Port=15
  wires:
  sim_data0/1 -> gain0/1
  gain0/1 -> bias0/1
  bias0/1 -> d0_ds0/1, d0_ds1/1, d0_ds2/1, d0_ds3/1
  d0_ds0/1 -> d0_del0/1
  d0_del0/1 -> xps_library_katadc_user_datai0/1, lt0_0/1, gt0_0/1
  xps_library_katadc_user_datai0/1 -> sign0_0/1, val0_0/1
  sign0_0/1 -> inv0_0/1
  inv0_0/1 -> concat0_0/1
  val0_0/1 -> concat0_0/2
  concat0_0/1 -> reinterpret0_0/1
  reinterpret0_0/1 -> data0_0/1
  d0_ds1/1 -> d0_del1/1
  d0_del1/1 -> xps_library_katadc_user_datai1/1, lt0_1/1, gt0_1/1
  xps_library_katadc_user_datai1/1 -> sign0_1/1, val0_1/1
  sign0_1/1 -> inv0_1/1
  inv0_1/1 -> concat0_1/1
  val0_1/1 -> concat0_1/2
  concat0_1/1 -> reinterpret0_1/1
  reinterpret0_1/1 -> data0_1/1
  d0_ds2/1 -> d0_del2/1
  d0_del2/1 -> xps_library_katadc_user_datai2/1, lt0_2/1, gt0_2/1
  xps_library_katadc_user_datai2/1 -> sign0_2/1, val0_2/1
  sign0_2/1 -> inv0_2/1
  inv0_2/1 -> concat0_2/1
  val0_2/1 -> concat0_2/2
  concat0_2/1 -> reinterpret0_2/1
  reinterpret0_2/1 -> data0_2/1
  d0_ds3/1 -> d0_del3/1
  d0_del3/1 -> xps_library_katadc_user_datai3/1, lt0_3/1, gt0_3/1
  xps_library_katadc_user_datai3/1 -> sign0_3/1, val0_3/1
  sign0_3/1 -> inv0_3/1
  inv0_3/1 -> concat0_3/1
  val0_3/1 -> concat0_3/2
  concat0_3/1 -> reinterpret0_3/1
  reinterpret0_3/1 -> data0_3/1
  lt0_0/1 -> logical0/1
  gt0_0/1 -> logical0/2
  lt0_1/1 -> logical0/3
  gt0_1/1 -> logical0/4
  lt0_2/1 -> logical0/5
  gt0_2/1 -> logical0/6
  lt0_3/1 -> logical0/7
  gt0_3/1 -> logical0/8
  logical0/1 -> xps_library_katadc_user_outofrange0/1
  xps_library_katadc_user_outofrange0/1 -> or0/1
  sim_data1/1 -> gain1/1
  gain1/1 -> bias1/1
  bias1/1 -> d1_ds0/1, d1_ds1/1, d1_ds2/1, d1_ds3/1
  d1_ds0/1 -> d1_del0/1
  d1_del0/1 -> xps_library_katadc_user_dataq0/1, lt1_0/1, gt1_0/1
  xps_library_katadc_user_dataq0/1 -> sign1_0/1, val1_0/1
  sign1_0/1 -> inv1_0/1
  inv1_0/1 -> concat1_0/1
  val1_0/1 -> concat1_0/2
  concat1_0/1 -> reinterpret1_0/1
  reinterpret1_0/1 -> data1_0/1
  d1_ds1/1 -> d1_del1/1
  d1_del1/1 -> xps_library_katadc_user_dataq1/1, lt1_1/1, gt1_1/1
  xps_library_katadc_user_dataq1/1 -> sign1_1/1, val1_1/1
  sign1_1/1 -> inv1_1/1
  inv1_1/1 -> concat1_1/1
  val1_1/1 -> concat1_1/2
  concat1_1/1 -> reinterpret1_1/1
  reinterpret1_1/1 -> data1_1/1
  d1_ds2/1 -> d1_del2/1
  d1_del2/1 -> xps_library_katadc_user_dataq2/1, lt1_2/1, gt1_2/1
  xps_library_katadc_user_dataq2/1 -> sign1_2/1, val1_2/1
  sign1_2/1 -> inv1_2/1
  inv1_2/1 -> concat1_2/1
  val1_2/1 -> concat1_2/2
  concat1_2/1 -> reinterpret1_2/1
  reinterpret1_2/1 -> data1_2/1
  d1_ds3/1 -> d1_del3/1
  d1_del3/1 -> xps_library_katadc_user_dataq3/1, lt1_3/1, gt1_3/1
  xps_library_katadc_user_dataq3/1 -> sign1_3/1, val1_3/1
  sign1_3/1 -> inv1_3/1
  inv1_3/1 -> concat1_3/1
  val1_3/1 -> concat1_3/2
  concat1_3/1 -> reinterpret1_3/1
  reinterpret1_3/1 -> data1_3/1
  lt1_0/1 -> logical1/1
  gt1_0/1 -> logical1/2
  lt1_1/1 -> logical1/3
  gt1_1/1 -> logical1/4
  lt1_2/1 -> logical1/5
  gt1_2/1 -> logical1/6
  lt1_3/1 -> logical1/7
  gt1_3/1 -> logical1/8
  logical1/1 -> xps_library_katadc_user_outofrange1/1
  xps_library_katadc_user_outofrange1/1 -> or1/1
  sim_sync/1 -> sync_ds0/1, sync_ds1/1, sync_ds2/1, sync_ds3/1
  sync_ds0/1 -> sync_del0/1
  sync_del0/1 -> xps_library_katadc_user_sync0/1
  xps_library_katadc_user_sync0/1 -> sync0/1
  sync_ds1/1 -> sync_del1/1
  sync_del1/1 -> xps_library_katadc_user_sync1/1
  xps_library_katadc_user_sync1/1 -> sync1/1
  sync_ds2/1 -> sync_del2/1
  sync_del2/1 -> xps_library_katadc_user_sync2/1
  xps_library_katadc_user_sync2/1 -> sync2/1
  sync_ds3/1 -> sync_del3/1
  sync_del3/1 -> xps_library_katadc_user_sync3/1
  xps_library_katadc_user_sync3/1 -> sync3/1
  sim_data_valid/1 -> xps_library_katadc_user_data_valid/1
  xps_library_katadc_user_data_valid/1 -> data_valid/1
  en0/1 -> slc0/1
  atten0/1 -> slc1/1
  slc1/1 -> inv0/1
  en1/1 -> slc2/1
  atten1/1 -> slc3/1
  slc3/1 -> inv1/1
  trigger/1 -> con/1
  slc0/1 -> con/4
  inv0/1 -> con/5
  slc2/1 -> con/2
  inv1/1 -> con/3
  con/1 -> reg/1, changed/2
  reg/1 -> changed/1, slc4/1
  slc4/1 -> cast0/1
  cast0/1 -> xps_library_katadc_gain_value/1
  changed/1 -> cast1/1
  cast1/1 -> xps_library_katadc_gain_load/1
